simulink model "Simscape_Drone_Model"  (R2025b)
settings: Solver=FixedStepAuto  StartTime=0.0  StopTime=10  RelTol=1e-6  EnableMultiTasking=on
undefined symbols (not defined in the file): Aero_On, Config, P, SimParams, SimscapeParams, X, Y, Z
libraries: sm_lib x89, nesl_utility x71, fl_lib x18, sdl_lib x8, slpidlib x4, batteryecm_lib x1
(part 1 of 5)
settings Model: Creator=Wombat_Simulator  LastModifiedBy=marku
settings SolverCC: ZeroCrossAlgorithm=Adaptive  PositivePriorityOrder=on  AutoInsertRateTranBlk=on
settings DataIOCC: SaveOutput=off  SaveTime=off
settings OptimizationCC: DefaultParameterBehavior=Inlined  EnhancedBackFolding=on  PassReuseOutputArgsAs=Individual arguments  ZeroExternalMemoryAtStartup=off  ZeroInternalMemoryAtStartup=off  MaxStackSize=64  OptimizeBlockOrder=speed  DifferentSizesBufferReuse=on  EfficientTunableParamExpr=on
settings DebuggingCC: IgnoredZcDiagnostic=none  ParameterTunabilityLossMsg=error
settings HardwareCC: ProdBitPerPointer=32.0  ProdBitPerSizeT=32.0  ProdBitPerPtrDiffT=32.0  ProdLargestAtomicInteger=Long  ProdLargestAtomicFloat=Double  ProdWordSize=32.0  ProdHWDeviceType=ARM Compatible->ARM Cortex-A (32-bit)
settings SFSimCC: MATLABDynamicMemAlloc=off
settings RTWCC: SystemTargetFile=ert.tlc  TemplateMakefile=ert_default_tmf  Description=Embedded Coder
settings CodeAppCC: ForceParamTrailComments=on  IgnoreCustomStorageClasses=off  OperatorAnnotations=on  SimulinkDataObjDesc=on  SFDataObjDesc=on  InsertBlockDesc=on
settings ERTTargetCC: ExtModeStaticAlloc=on  InlinedParameterPlacement=Hierarchical  ERTCustomFileTemplate=example_file_process.tlc  SupportNonInlinedSFcns=on
settings ExplorerConfigSet: InternalSimMechanicsExplorerSettings=|
  | <ExplorerConfiguration>
  | 
  |   <canonicalview>default</canonicalview>
  | 
  |   <TilePanel>
  |     <TileInfo>
  |       <Tiles Columns="1" Count="1" Height="1184" Rows="1" Width="2103">
  |         <Row Weight="1"/>
  |         <Column Weight="1"/>
  |         <Tile Height="1" Width="1" X="0" Y="0"/>
  |       </Tiles>
  |     </TileInfo>
  |     <SceneInfo>
  |       <SceneViewer>
  |         <IsThisViewStd>
  |           <IsStandardView>off</IsStandardView>
  |           <StandardViewName>Front</StandardViewName>
  |         </IsThisViewStd>
  |         <BGColor>
  |           <R>1</R>
  |           <G>1</G>
  |           <B>1</B>
  |           <A>1</A>
  |         </BGColor>
  |         <Camera>
  |           <DoPerspective>on</DoPerspective>
  |           <Position>
  |             <X>-0.70406999999999997</X>
  |             <Y>24.994199999999999</Y>
  |             <Z>0.5675</Z>
  |           </Position>
  |           <Center>
  |             <X>-0.56381999999999999</X>
  |             <Y>27.990919999999999</Y>
  |             <Z>-0.43248999999999999</Z>
  |           </Center>
  |           <Up>
  |             <X>0.014783513727254149</X>
  |             <Y>0.31587915334571876</Y>
  |             <Z>0.94868425105694032</Z>
  |           </Up>
  |           <XLim>1.4745942901489864</XLim>
  |           <YLim>1.4745942901489864</YLim>
  |           <ViewLimDist>0.01</ViewLimDist>
  |         </Camera>
  |       </SceneViewer>
  |     </SceneInfo>
  |   </TilePanel>
  | 
  |   <MechEditorPanel>
  |     <GfxPanelCameraMap>
  |       <MapElement CameraMLId="Camera1" GfxPanelIndex="0"/>
  |     </GfxPanelCameraMap>
  |     <Cameras>
  |       <Camera>
  |         <Id>Camera1</Id>
  |         <Value>
  |           <Name>Camera1</Name>
  |           <NativeCamera>
  |             <PositionTrackingFeature>Drone_Mechanics.x6DOF.Camera_frame.F</PositionTrackingFeature>
  |             <CenterTrackingFeature>Drone_Mechanics.x6DOF.CoB</CenterTrackingFeature>
  |             <UpVectorTrackingFeature>Drone_Mechanics.Ground.NED</UpVectorTrackingFeature>
  |             <CenterTrackingOrigin>on</CenterTrackingOrigin>
  |             <UpVectorTrackingDirection>-Z</UpVectorTrackingDirection>
  |           </NativeCamera>
  |         </Value>
  |       </Camera>
  |     </Cameras>
  |     <VideoCreator>
  |       <IncludeTiles>All</IncludeTiles>
  |       <IncludeTime>on</IncludeTime>
  |       <IncludeWorldFrame>off</IncludeWorldFrame>
  |       <PlaybackSpeedRatio>1</PlaybackSpeedRatio>
  |       <FrameRate>30</FrameRate>
  |       <FrameSize>auto</FrameSize>
  |       <VideoFormat>UncompressedAVI</VideoFormat>
  |     </VideoCreator>
  |   </MechEditorPanel>
  | 
  |   <PlaybackSettings>
  |     <PlaybackSpeedFactor>1</PlaybackSpeedFactor>
  |   </PlaybackSettings>
  | 
  | </ExplorerConfiguration>

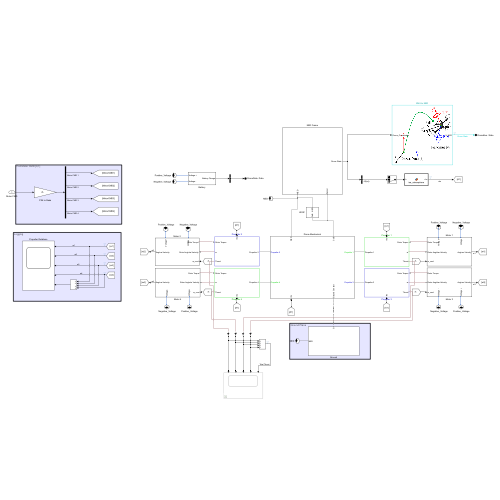
[thumbnail: Simulink's stored preview of the top-level diagram]
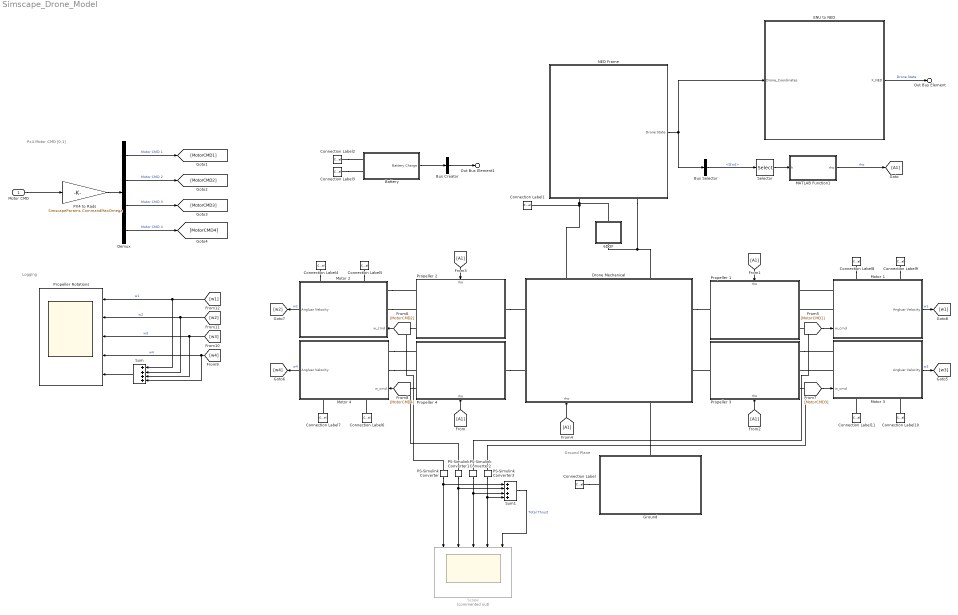
== system Simscape_Drone_Model ==
  note: Logging
  note: Ground Plane
  note: Px4 Motor CMD [0,1]
  Motor CMD : Inport
  6DOF : Subsystem
  Battery : Subsystem
  Bus Creator : BusCreator  Inputs=1
  Bus Selector : BusSelector  OutputSignals=S[m]
  Connection Label : ConnectionLabel  Label=NED
  Connection Label1 : ConnectionLabel  Label=NED
  Connection Label{2,4,6,8,10} (5 alike) : ConnectionLabel  Tag=simrfV2util1/Connection Label  Label=Positive_Voltage
  Connection Label{3,5,7,9,11} (5 alike) : ConnectionLabel  Tag=simrfV2util1/Connection Label  Label=Negative_Voltage
  Demux : Demux
  Drone Mechanical : Subsystem
      settings: PortSchema="{\"entries\":[{\"content\":{\"sides\":[{\"content\":{\"connectorIds\":[\"LConn1\",\"LConn2\"]},\"type\":\"ConnectorPlacement.EquallySpacedRectSide\",\"uuid\":\"5cc608d4-ddbf-4612-8fb9-2660b822e984\"},{\"content\":{\"connectorIds\":[\"RConn1\",\"RConn2\"],\"side\":\"RIGHT\"},\"type\":\"ConnectorPlacement.EquallySpacedRectSide\",\"uuid\":\"5a60fbc0-e4d8-4b3c-ab9e-99a47e43b410\"},{\"content\":{\"connectorIds\":[\"LConn3\",\"LConn4\"],\"side\":\"TOP\"},\"type\":\"ConnectorPlacement.EquallySpacedRectSide\",\"uuid\":\"82070e07-6e43-48ae-84e2-45e211cce44a\"},{\"content\":{\"connectorIds\":[\"In1\",\"RConn3\"],\"side\":\"BOTTOM\"},\"type\":\"ConnectorPlacement.EquallySpacedRectSide\",\"uuid\":\"b93c099a-11e8-4ef2-b906-259b9ea4f5ed\"}]},\"type\":\"ConnectorPlacement.EquallySpacedConnector\",\"uuid\":\"249715e8-12e0-4eae-8212-72e654615a84\"}],\"packageUris\":[\"http://schema.mathworks.com/mf0/Connector/R2020b\"],\"version\":\"1.0\"}"
  ENU to NED : Subsystem
      mask Display: image('World Frame Conversion.png');
  Ground : Subsystem
      settings: PortSchema="{\"entries\":[{\"content\":{\"sides\":[{\"content\":{\"connectorIds\":[\"LConn1\"]},\"type\":\"ConnectorPlacement.EquallySpacedRectSide\",\"uuid\":\"2a080899-5da5-46e1-952c-d17a92ba1a8b\"},{\"content\":{\"side\":\"RIGHT\"},\"type\":\"ConnectorPlacement.EquallySpacedRectSide\",\"uuid\":\"3b513f94-3d5d-4528-8948-7d09eae76d3d\"},{\"content\":{\"connectorIds\":[\"LConn2\"],\"side\":\"TOP\"},\"type\":\"ConnectorPlacement.EquallySpacedRectSide\",\"uuid\":\"f80b446f-13e5-4ac1-9992-a76049c3ec7c\"}]},\"type\":\"ConnectorPlacement.EquallySpacedConnector\",\"uuid\":\"dd2a473b-5f76-4ac8-b09e-9b626a8e8601\"}],\"packageUris\":[\"http://schema.mathworks.com/mf0/Connector/R2020b\"],\"version\":\"1.0\"}"
  MATLAB Function1 : MATLAB Function  TreatAsAtomicUnit=on
  Motor 1 : Subsystem
      settings: PortSchema="{\"entries\":[{\"content\":{\"sides\":[{\"content\":{\"connectorIds\":[\"LConn1\",\"LConn2\",\"In1\"]},\"type\":\"ConnectorPlacement.EquallySpacedRectSide\",\"uuid\":\"33dc3d2f-8968-4f36-a17e-891381f68888\"},{\"content\":{\"connectorIds\":[\"Out1\"],\"side\":\"RIGHT\"},\"type\":\"ConnectorPlacement.EquallySpacedRectSide\",\"uuid\":\"508781b7-b827-4221-88b7-22df8b6754af\"},{\"content\":{\"connectorIds\":[\"LConn3\",\"LConn4\"],\"side\":\"TOP\"},\"type\":\"ConnectorPlacement.EquallySpacedRectSide\",\"uuid\":\"a75d12a6-d4ec-4522-becc-e9bbf7a7aed5\"}]},\"type\":\"ConnectorPlacement.EquallySpacedConnector\",\"uuid\":\"704cc29a-e448-45b3-ab6f-6d8987c901fd\"}],\"packageUris\":[\"http://schema.mathworks.com/mf0/Connector/R2020b\"],\"version\":\"1.0\"}"
  Motor 2 : Subsystem
      settings: PortSchema="{\"entries\":[{\"content\":{\"sides\":[{\"content\":{\"connectorIds\":[\"LConn1\",\"LConn2\",\"In1\"]},\"type\":\"ConnectorPlacement.EquallySpacedRectSide\",\"uuid\":\"ab24fea9-a927-40b5-bce5-f99779c8987a\"},{\"content\":{\"connectorIds\":[\"Out1\"],\"side\":\"RIGHT\"},\"type\":\"ConnectorPlacement.EquallySpacedRectSide\",\"uuid\":\"e5fff93c-3e20-4c5e-b15c-bef5c876d182\"},{\"content\":{\"connectorIds\":[\"LConn3\",\"LConn4\"],\"side\":\"TOP\"},\"type\":\"ConnectorPlacement.EquallySpacedRectSide\",\"uuid\":\"e8b793e7-5ef5-4a63-a387-509c68cd63b8\"}]},\"type\":\"ConnectorPlacement.EquallySpacedConnector\",\"uuid\":\"3d309d3b-67ba-4e78-84bc-eb68d5ca7651\"}],\"packageUris\":[\"http://schema.mathworks.com/mf0/Connector/R2020b\"],\"version\":\"1.0\"}"
  Motor 3 : Subsystem
      settings: PortSchema="{\"entries\":[{\"content\":{\"sides\":[{\"content\":{\"connectorIds\":[\"LConn1\",\"LConn2\",\"In1\"]},\"type\":\"ConnectorPlacement.EquallySpacedRectSide\",\"uuid\":\"33dc3d2f-8968-4f36-a17e-891381f68888\"},{\"content\":{\"connectorIds\":[\"Out1\"],\"side\":\"RIGHT\"},\"type\":\"ConnectorPlacement.EquallySpacedRectSide\",\"uuid\":\"508781b7-b827-4221-88b7-22df8b6754af\"},{\"content\":{\"side\":\"TOP\"},\"type\":\"ConnectorPlacement.EquallySpacedRectSide\",\"uuid\":\"a75d12a6-d4ec-4522-becc-e9bbf7a7aed5\"},{\"content\":{\"connectorIds\":[\"RConn1\",\"RConn2\"],\"side\":\"BOTTOM\"},\"type\":\"ConnectorPlacement.EquallySpacedRectSide\",\"uuid\":\"c496d817-d9a7-4570-9947-2d46969d8890\"}]},\"type\":\"ConnectorPlacement.EquallySpacedConnector\",\"uuid\":\"704cc29a-e448-45b3-ab6f-6d8987c901fd\"}],\"packageUris\":[\"http://schema.mathworks.com/mf0/Connector/R2020b\"],\"version\":\"1.0\"}"
  Motor 4 : Subsystem
      settings: PortSchema="{\"entries\":[{\"content\":{\"sides\":[{\"content\":{\"connectorIds\":[\"In1\",\"LConn1\",\"LConn2\"]},\"type\":\"ConnectorPlacement.EquallySpacedRectSide\",\"uuid\":\"e00824c0-1364-4e77-bc63-912ddc8593ef\"},{\"content\":{\"connectorIds\":[\"Out1\"],\"side\":\"RIGHT\"},\"type\":\"ConnectorPlacement.EquallySpacedRectSide\",\"uuid\":\"0a7636ad-9e2c-497e-9c6a-850c3925dcad\"},{\"content\":{\"connectorIds\":[\"LConn3\",\"LConn4\"],\"side\":\"TOP\"},\"type\":\"ConnectorPlacement.EquallySpacedRectSide\",\"uuid\":\"0b319ad1-75e7-4a0f-96b2-2e5629eeb7ef\"}]},\"type\":\"ConnectorPlacement.EquallySpacedConnector\",\"uuid\":\"157f13eb-3591-4c9f-b2fb-1cc94b60842e\"}],\"packageUris\":[\"http://schema.mathworks.com/mf0/Connector/R2020b\"],\"version\":\"1.0\"}"
  NED Frame : Subsystem
      settings: PortSchema="{\"entries\":[{\"content\":{\"sides\":[{\"content\":{},\"type\":\"ConnectorPlacement.EquallySpacedRectSide\",\"uuid\":\"2f7c4040-ad72-4a4e-bca0-490c9a3edb01\"},{\"content\":{\"connectorIds\":[\"RConn1\",\"RConn2\"],\"side\":\"RIGHT\"},\"type\":\"ConnectorPlacement.EquallySpacedRectSide\",\"uuid\":\"95b4bfac-22e1-4427-9780-ec2091d8174e\"},{\"content\":{\"side\":\"TOP\"},\"type\":\"ConnectorPlacement.EquallySpacedRectSide\",\"uuid\":\"6fc8ef3e-afe1-420d-8beb-cc9354b2a683\"},{\"content\":{\"connectorIds\":[\"Out1\"],\"side\":\"BOTTOM\"},\"type\":\"ConnectorPlacement.EquallySpacedRectSide\",\"uuid\":\"fddcf54a-6ad4-4366-b56a-6290dfac1197\"}]},\"type\":\"ConnectorPlacement.EquallySpacedConnector\",\"uuid\":\"4cba3fee-e392-4a87-a4f1-4e77f5fdcd83\"}],\"packageUris\":[\"http://schema.mathworks.com/mf0/Connector/R2020b\"],\"version\":\"1.0\"}"
  PS-Simulink Converter{,1..3} (4 alike) : nesl_utility/PS-Simulink Converter  PhysicalDomain=network_engine_domain  SubClassName=ps_output  LeftPortType=input  RightPortType=output  PseudoPeriodic=off  Frequencies=[]  VectorFormat=inherit  Unit=inherit  AffineConversion=off
  PX4 to Rads : Gain  Gain=SimscapeParams.CommandMaxOmega
  Propeller 1 : Subsystem
      settings: PortSchema="{\"entries\":[{\"content\":{\"sides\":[{\"content\":{\"connectorIds\":[\"LConn1\"]},\"type\":\"ConnectorPlacement.EquallySpacedRectSide\",\"uuid\":\"a11f93c9-60b9-4980-b5fb-77cb9445bf15\"},{\"content\":{\"connectorIds\":[\"RConn1\",\"RConn2\",\"RConn3\"],\"side\":\"RIGHT\"},\"type\":\"ConnectorPlacement.EquallySpacedRectSide\",\"uuid\":\"b77a8a2e-4ab8-482f-9f6d-d9ab9ea7b696\"},{\"content\":{\"connectorIds\":[\"In1\"],\"side\":\"TOP\"},\"type\":\"ConnectorPlacement.EquallySpacedRectSide\",\"uuid\":\"fb34fa6b-cd57-4423-95d5-7f2443420811\"}]},\"type\":\"ConnectorPlacement.EquallySpacedConnector\",\"uuid\":\"b83f6b43-9a9e-4fc8-9a49-e0da42a3bbd0\"}],\"packageUris\":[\"http://schema.mathworks.com/mf0/Connector/R2020b\"],\"version\":\"1.0\"}"
  Propeller 2 : Subsystem
      settings: PortSchema="{\"entries\":[{\"content\":{\"sides\":[{\"content\":{\"connectorIds\":[\"LConn1\"]},\"type\":\"ConnectorPlacement.EquallySpacedRectSide\",\"uuid\":\"a11f93c9-60b9-4980-b5fb-77cb9445bf15\"},{\"content\":{\"connectorIds\":[\"RConn1\",\"RConn2\",\"RConn3\"],\"side\":\"RIGHT\"},\"type\":\"ConnectorPlacement.EquallySpacedRectSide\",\"uuid\":\"b77a8a2e-4ab8-482f-9f6d-d9ab9ea7b696\"},{\"content\":{\"connectorIds\":[\"In1\"],\"side\":\"TOP\"},\"type\":\"ConnectorPlacement.EquallySpacedRectSide\",\"uuid\":\"fb34fa6b-cd57-4423-95d5-7f2443420811\"},{\"content\":{\"side\":\"BOTTOM\"},\"type\":\"ConnectorPlacement.EquallySpacedRectSide\",\"uuid\":\"49b1b310-8b7b-4cf8-a23d-4dd8be08c88f\"}]},\"type\":\"ConnectorPlacement.EquallySpacedConnector\",\"uuid\":\"b83f6b43-9a9e-4fc8-9a49-e0da42a3bbd0\"}],\"packageUris\":[\"http://schema.mathworks.com/mf0/Connector/R2020b\"],\"version\":\"1.0\"}"
  Propeller 3 : Subsystem
      settings: PortSchema="{\"entries\":[{\"content\":{\"sides\":[{\"content\":{\"connectorIds\":[\"LConn1\"]},\"type\":\"ConnectorPlacement.EquallySpacedRectSide\",\"uuid\":\"a11f93c9-60b9-4980-b5fb-77cb9445bf15\"},{\"content\":{\"connectorIds\":[\"RConn1\",\"RConn2\",\"RConn3\"],\"side\":\"RIGHT\"},\"type\":\"ConnectorPlacement.EquallySpacedRectSide\",\"uuid\":\"b77a8a2e-4ab8-482f-9f6d-d9ab9ea7b696\"},{\"content\":{\"side\":\"TOP\"},\"type\":\"ConnectorPlacement.EquallySpacedRectSide\",\"uuid\":\"fb34fa6b-cd57-4423-95d5-7f2443420811\"},{\"content\":{\"connectorIds\":[\"In1\"],\"side\":\"BOTTOM\"},\"type\":\"ConnectorPlacement.EquallySpacedRectSide\",\"uuid\":\"7aad20ae-aa9d-4d5e-81ba-52dbfeaf9214\"}]},\"type\":\"ConnectorPlacement.EquallySpacedConnector\",\"uuid\":\"b83f6b43-9a9e-4fc8-9a49-e0da42a3bbd0\"}],\"packageUris\":[\"http://schema.mathworks.com/mf0/Connector/R2020b\"],\"version\":\"1.0\"}"
  Propeller 4 : Subsystem
      settings: PortSchema="{\"entries\":[{\"content\":{\"sides\":[{\"content\":{\"connectorIds\":[\"LConn1\"]},\"type\":\"ConnectorPlacement.EquallySpacedRectSide\",\"uuid\":\"a11f93c9-60b9-4980-b5fb-77cb9445bf15\"},{\"content\":{\"connectorIds\":[\"RConn1\",\"RConn2\",\"RConn3\"],\"side\":\"RIGHT\"},\"type\":\"ConnectorPlacement.EquallySpacedRectSide\",\"uuid\":\"b77a8a2e-4ab8-482f-9f6d-d9ab9ea7b696\"},{\"content\":{\"side\":\"TOP\"},\"type\":\"ConnectorPlacement.EquallySpacedRectSide\",\"uuid\":\"fb34fa6b-cd57-4423-95d5-7f2443420811\"},{\"content\":{\"connectorIds\":[\"In1\"],\"side\":\"BOTTOM\"},\"type\":\"ConnectorPlacement.EquallySpacedRectSide\",\"uuid\":\"82da3900-16a5-458e-a9d2-86e2be3a3c24\"}]},\"type\":\"ConnectorPlacement.EquallySpacedConnector\",\"uuid\":\"b83f6b43-9a9e-4fc8-9a49-e0da42a3bbd0\"}],\"packageUris\":[\"http://schema.mathworks.com/mf0/Connector/R2020b\"],\"version\":\"1.0\"}"
  Propeller Rotations : Scope  NumInputPorts=5
      settings: ActiveDisplayYMinimum=-108.37040231135038  ActiveDisplayYMaximum=951.06085463645354
  Scope : Scope  Commented=on  NumInputPorts=5
      settings: ActiveDisplayYMinimum=-798.82748260843846  ActiveDisplayYMaximum=139.02483072762607  DataLoggingVariableName=ScopeData5
  Selector : Selector  InputPortWidth=3  IndexOptions=Index vector (dialog)  Indices=[3]  OutputSizes=1
  Sum : Sum  Inputs=++++
  Sum1 : Sum  Inputs=++++
  Out Bus Element1 : Outport  PortName=DroneData  Element=Data
  Out Bus Element : Outport  Port=2  PortName=DroneBus  Element=State
  wires:
  MATLAB Function1/1(rho) -> [A1]  "rho"
  [A1] -> Propeller 4/1(rho)
  [A1] -> Propeller 1/1(rho)
  [A1] -> Propeller 3/1(rho)
  [A1] -> Propeller 2/1(rho)
  [A1] -> Drone Mechanical/1(rho)
  Sum/1 -> Propeller Rotations/5
  NED Frame/1(Drone State) -> ENU to NED/1(Drone_Coordinates), Bus Selector/1
  Demux/1 -> [MotorCMD1]  "Motor CMD 1"
  [MotorCMD1] -> Motor 1/1(w_cmd)
  Demux/2 -> [MotorCMD2]  "Motor CMD 2"
  [MotorCMD2] -> Motor 2/1(w_cmd)
  Demux/3 -> [MotorCMD3]  "Motor CMD 3"
  [MotorCMD3] -> Motor 3/1(w_cmd)
  Demux/4 -> [MotorCMD4]  "Motor CMD 4"
  [MotorCMD4] -> Motor 4/1(w_cmd)
  Selector/1 -> MATLAB Function1/1(h)
  Bus Selector/1 -> Selector/1  "<S[m]>"
  Battery/1(Battery Charge) -> Bus Creator/1
  Bus Creator/1 -> Out Bus Element1/1
  ENU to NED/1(X_NED) -> Out Bus Element/1  "Drone State"
  PX4 to Rads/1 -> Demux/1
  Motor 3/1(Angluar Velocity) -> [w3]  "w3"
  [w3] -> Propeller Rotations/3, Sum/3  "w3"
  Motor 4/1(Angluar Velocity) -> [w4]  "w4"
  [w4] -> Propeller Rotations/4, Sum/4  "w4"
  Motor 2/1(Angluar Velocity) -> [w2]  "w2"
  [w2] -> Propeller Rotations/2, Sum/2  "w2"
  Motor 1/1(Angluar Velocity) -> [w1]  "w1"
  [w1] -> Propeller Rotations/1, Sum/1  "w1"
  PS-Simulink Converter/1 -> Scope/1, Sum1/1
  PS-Simulink Converter1/1 -> Scope/2, Sum1/2
  PS-Simulink Converter2/1 -> Scope/3, Sum1/3
  PS-Simulink Converter3/1 -> Scope/4, Sum1/4
  Motor CMD/1 -> PX4 to Rads/1
  Sum1/1 -> Scope/5  "Total Thrust"
  connections:
  6DOF/LConn1 -- Connection Label1/LConn1 -- Drone Mechanical/LConn3 -- NED Frame/RConn1
  6DOF/RConn1 -- NED Frame/RConn2 -- Drone Mechanical/LConn4
  Motor 1/LConn2 -- Propeller 1/RConn2
  Propeller 3/LConn1 -- Drone Mechanical/RConn2
  Propeller 3/RConn1 -- Motor 3/LConn1
  Motor 2/LConn1 -- Propeller 2/RConn1
  Connection Label/LConn1 -- Ground/LConn1
  Propeller 2/LConn1 -- Drone Mechanical/LConn1
  Motor 2/LConn2 -- Propeller 2/RConn2
  Propeller 4/LConn1 -- Drone Mechanical/LConn2
  Motor 1/LConn1 -- Propeller 1/RConn1
  Motor 4/LConn1 -- Propeller 4/RConn2
  Ground/LConn2 -- Drone Mechanical/RConn3
  Drone Mechanical/RConn1 -- Propeller 1/LConn1
  Motor 4/LConn2 -- Propeller 4/RConn1
  Motor 3/LConn2 -- Propeller 3/RConn2
  Connection Label2/LConn1 -- Battery/LConn1
  Connection Label3/LConn1 -- Battery/LConn2
  Connection Label4/LConn1 -- Motor 2/LConn4
  Connection Label5/LConn1 -- Motor 2/LConn3
  Connection Label6/LConn1 -- Motor 4/LConn3
  Connection Label7/LConn1 -- Motor 4/LConn4
  Connection Label8/LConn1 -- Motor 1/LConn3
  Connection Label9/LConn1 -- Motor 1/LConn4
  Connection Label11/LConn1 -- Motor 3/RConn1
  Connection Label10/LConn1 -- Motor 3/RConn2
  PS-Simulink Converter/LConn1 -- Propeller 2/RConn3
  PS-Simulink Converter1/LConn1 -- Propeller 4/RConn3
  PS-Simulink Converter2/LConn1 -- Propeller 1/RConn3
  PS-Simulink Converter3/LConn1 -- Propeller 3/RConn3

== system Simscape_Drone_Model/6DOF ==
  6-DOF Joint : sm_lib/Joints/6-DOF Joint  JointMode=Normal  CompositeWrenchDir=FollowerOnBase  CompositeWrenchFrame=BaseFrame  SenseConstraintForce=off  SenseConstraintTorque=off  SenseTotalForce=off  SenseTotalTorque=off  PxPositionTargetSpecify=off  PxPositionTargetPriority=High  PxPositionTargetValue=0  PxPositionTargetValueUnits=m  PxVelocityTargetSpecify=off  PxVelocityTargetPriority=High  PxVelocityTargetValue=0  PxVelocityTargetValueUnits=m/s  PxEquilibriumPosition=0  PxEquilibriumPositionUnits=m  PxSpringStiffness=0  PxSpringStiffnessUnits=N/m  PxDampingCoefficient=0  PxDampingCoefficientUnits=N/(m/s)  PxLowerLimitSpecify=off  PxLowerLimitBound=-1  PxLowerLimitBoundUnits=m  PxLowerLimitStiffness=1e6  PxLowerLimitStiffnessUnits=N/m  PxLowerLimitDamping=1e3  PxLowerLimitDampingUnits=N/(m/s)  PxLowerLimitTransitionRegionWidth=1e-4  PxLowerLimitTransitionRegionWidthUnits=m  PxUpperLimitSpecify=off  PxUpperLimitBound=1  PxUpperLimitBoundUnits=m  PxUpperLimitStiffness=1e6  PxUpperLimitStiffnessUnits=N/m  PxUpperLimitDamping=1e3  PxUpperLimitDampingUnits=N/(m/s)  PxUpperLimitTransitionRegionWidth=1e-4  PxUpperLimitTransitionRegionWidthUnits=m  PxTorqueActuationMode=NoTorque  PxMotionActuationMode=ComputedMotion  PxSensePosition=off  PxSenseVelocity=off  PxSenseAcceleration=off  PxSenseTorqueForce=off  PxSenseLowerLimitTorqueForce=off  PxSenseUpperLimitTorqueForce=off  PyPositionTargetSpecify=off  PyPositionTargetPriority=High  PyPositionTargetValue=0  PyPositionTargetValueUnits=m  PyVelocityTargetSpecify=off  PyVelocityTargetPriority=High  PyVelocityTargetValue=0  PyVelocityTargetValueUnits=m/s  PyEquilibriumPosition=0  PyEquilibriumPositionUnits=m  PySpringStiffness=0  PySpringStiffnessUnits=N/m  PyDampingCoefficient=0  PyDampingCoefficientUnits=N/(m/s)  PyLowerLimitSpecify=off  PyLowerLimitBound=-1  PyLowerLimitBoundUnits=m  PyLowerLimitStiffness=1e6  PyLowerLimitStiffnessUnits=N/m  PyLowerLimitDamping=1e3  PyLowerLimitDampingUnits=N/(m/s)  PyLowerLimitTransitionRegionWidth=1e-4  PyLowerLimitTransitionRegionWidthUnits=m  PyUpperLimitSpecify=off  PyUpperLimitBound=1  PyUpperLimitBoundUnits=m  PyUpperLimitStiffness=1e6  PyUpperLimitStiffnessUnits=N/m  PyUpperLimitDamping=1e3  PyUpperLimitDampingUnits=N/(m/s)  PyUpperLimitTransitionRegionWidth=1e-4  PyUpperLimitTransitionRegionWidthUnits=m  PyTorqueActuationMode=NoTorque  PyMotionActuationMode=ComputedMotion  PySensePosition=off  PySenseVelocity=off  PySenseAcceleration=off  PySenseTorqueForce=off  PySenseLowerLimitTorqueForce=off  PySenseUpperLimitTorqueForce=off  PzPositionTargetSpecify=off  PzPositionTargetPriority=High  PzPositionTargetValue=-500  PzPositionTargetValueUnits=m  PzVelocityTargetSpecify=off  PzVelocityTargetPriority=High  PzVelocityTargetValue=0  PzVelocityTargetValueUnits=m/s  PzEquilibriumPosition=0  PzEquilibriumPositionUnits=m  PzSpringStiffness=0  PzSpringStiffnessUnits=N/m  PzDampingCoefficient=0  PzDampingCoefficientUnits=N/(m/s)  PzLowerLimitSpecify=off  PzLowerLimitBound=-1  PzLowerLimitBoundUnits=m  PzLowerLimitStiffness=1e6  PzLowerLimitStiffnessUnits=N/m  PzLowerLimitDamping=1e3  PzLowerLimitDampingUnits=N/(m/s)  PzLowerLimitTransitionRegionWidth=1e-4  PzLowerLimitTransitionRegionWidthUnits=m  PzUpperLimitSpecify=off  PzUpperLimitBound=1  PzUpperLimitBoundUnits=m  PzUpperLimitStiffness=1e6  PzUpperLimitStiffnessUnits=N/m  PzUpperLimitDamping=1e3  PzUpperLimitDampingUnits=N/(m/s)  PzUpperLimitTransitionRegionWidth=1e-4  PzUpperLimitTransitionRegionWidthUnits=m  PzTorqueActuationMode=NoTorque  PzMotionActuationMode=ComputedMotion  PzSensePosition=off  PzSenseVelocity=off  PzSenseAcceleration=off  PzSenseTorqueForce=off  PzSenseLowerLimitTorqueForce=off  PzSenseUpperLimitTorqueForce=off  SphPositionTargetSpecify=off  SphPositionTargetPriority=High  SphPositionTargetRotationMethod=None  SphPositionTargetFollAlignAxisA=+X  SphPositionTargetBaseAlignAxisA=+Y  SphPositionTargetFollAlignAxisB=+Y  SphPositionTargetBaseAlignAxisB=+Z  SphPositionTargetRotationStandardAxis=+Z  SphPositionTargetRotationAngle=0  SphPositionTargetRotationAngleUnits=deg  SphPositionTargetRotationArbitraryAxis=[0 0 1]  SphPositionTargetRotationSequenceAxes=FollowerAxes  SphPositionTargetRotationSequence=XYX  SphPositionTargetRotationSequenceAngles=[0 0 0]  SphPositionTargetRotationSequenceAnglesUnits=deg  SphPositionTargetRotationMatrix=[1 0 0;0 1 0;0 0 1]  SphPositionTargetQuaternion=[1 0 0 0]  SphVelocityTargetSpecify=off  SphVelocityTargetPriority=High  SphVelocityTargetValue=[0 0 0]  SphVelocityTargetValueUnits=deg/s  SphVelocityTargetInFollowerFrame=on  SphEqPosRotationMethod=None  SphEqPosFollAlignAxisA=+X  SphEqPosBaseAlignAxisA=+Y  SphEqPosFollAlignAxisB=+Y  SphEqPosBaseAlignAxisB=+Z  SphEqPosRotationStandardAxis=+Z  SphEqPosRotationAngle=0  SphEqPosRotationAngleUnits=deg  SphEqPosRotationArbitraryAxis=[0 0 1]  SphEqPosRotationSequenceAxes=FollowerAxes  SphEqPosRotationSequence=XYX  SphEqPosRotationSequenceAngles=[0 0 0]  SphEqPosRotationSequenceAnglesUnits=deg  SphEqPosRotationMatrix=[1 0 0;0 1 0;0 0 1]  SphEqPosQuaternion=[1 0 0 0]  SphSpringStiffness=0  SphSpringStiffnessUnits=N*m/deg  SphDampingCoefficient=0  SphDampingCoefficientUnits=N*m/(deg/s)  SphLowerLimitSpecify=off  SphLowerLimitBound=15  SphLowerLimitBoundUnits=deg  SphLowerLimitStiffness=1e4  SphLowerLimitStiffnessUnits=N*m/deg  SphLowerLimitDamping=10  SphLowerLimitDampingUnits=N*m/(deg/s)  SphLowerLimitTransitionRegionWidth=0.1  SphLowerLimitTransitionRegionWidthUnits=deg  SphUpperLimitSpecify=off  SphUpperLimitBound=45  SphUpperLimitBoundUnits=deg  SphUpperLimitStiffness=1e4  SphUpperLimitStiffnessUnits=N*m/deg  SphUpperLimitDamping=10  SphUpperLimitDampingUnits=N*m/(deg/s)  SphUpperLimitTransitionRegionWidth=0.1  SphUpperLimitTransitionRegionWidthUnits=deg  SphTorqueActuationMode=NoTorque  SphActuateTorqueX=off  SphActuateTorqueY=off  SphActuateTorqueZ=off  SphActuateTorque=off  SphActuationFrame=BaseFrame  SphSensePosition=off  SphSenseVelocityX=off  SphSenseVelocityY=off  SphSenseVelocityZ=off  SphSenseVelocity=off  SphSenseAccelerationX=off  SphSenseAccelerationY=off  SphSenseAccelerationZ=off  SphSenseAcceleration=off  SphSenseLowerLimitTorqueMag=off  SphSenseUpperLimitTorqueMag=off  SphSensingFrame=BaseFrame
  Camera frame : sm_lib/Frames and Transforms/Rigid Transform  Commented=on  RotationMethod=RotationSequence  FollAlignAxisA=+X  BaseAlignAxisA=+Y  FollAlignAxisB=+Y  BaseAlignAxisB=+Z  RotationStandardAxis=+Z  RotationAngle=0  RotationAngleUnits=deg  RotationArbitraryAxis=[0 0 1]  RotationSequenceAxes=BaseAxes  RotationSequence=XYZ  RotationSequenceAngles=[0 0 0]  RotationSequenceAnglesUnits=deg  RotationMatrix=[1 0 0;0 1 0;0 0 1]  Quaternion=[1 0 0 0]  TranslationMethod=Cartesian  TranslationCartesianOffset=[-5 0 -2]  TranslationCartesianOffsetUnits=m  TranslationStandardAxis=+Z  TranslationStandardOffset=0  TranslationStandardOffsetUnits=m  TranslationROffset=0  TranslationROffsetUnits=m  TranslationThetaOffset=0  TranslationThetaOffsetUnits=deg  TranslationZOffset=0  TranslationZOffsetUnits=m
  Inertia1 : sm_lib/Body Elements/Inertia  Commented=on  InertiaType=PointMass  Mass=0.00000001  MassUnits=kg  CenterOfMass=[0 0 0]  CenterOfMassUnits=m  MomentsOfInertia=[1 1 1]  MomentsOfInertiaUnits=kg*m^2  ProductsOfInertia=[0 0 0]  ProductsOfInertiaUnits=kg*m^2  GraphicType=None  MarkerShape=Inertia  MarkerSize=20  GraphicVisPropType=SimpleVisualProperties  GraphicDiffuseColor=[0.5 0.5 0.5]  GraphicOpacity=1  GraphicSpecularColor=[0.5 0.5 0.5 1.0]  GraphicAmbientColor=[0.15 0.15 0.15 1.0]  GraphicEmissiveColor=[0.0 0.0 0.0 1.0]  GraphicShininess=75
  NED : PMIOPort  Side=Left
  CoB : PMIOPort  Port=2  Side=Right
  connections:
  Inertia1/RConn1 -- Camera frame/RConn1
  Camera frame/LConn1 -- 6-DOF Joint/RConn1 -- CoB/RConn1
  6-DOF Joint/LConn1 -- NED/RConn1

== system Simscape_Drone_Model/Battery ==
  Battery1 : batteryecm_lib/Battery  Vnom=21.6 V  prm_dir=simscape.enum.battery.prm_dir.disabled  R1_dis=2 Ohm  R1_ch=2 Ohm  R1=0.01 Ohm  prm_AH=simscape.enum.battery.prm_AH.infinite  AH=50 A*hr  V1=11.5 V  AH1=25 A*hr  prm_R2=simscape.enum.battery.prm_R2.disabled  R2=2000 Ohm  Tmeas=298.15 K  charge_measurement_port=simscape.enum.battery.enable.yes  prm_dyn=simscape.enum.battery.prm_dyn.off  Rp1=0.005 Ohm  tau1=30 s  Rp2=0.005 Ohm  tau2=30 s  Rp3=0.005 Ohm  tau3=30 s  Rp4=0.005 Ohm  tau4=30 s  Rp5=0.005 Ohm  tau5=30 s  prm_fade=simscape.enum.battery.prm_fade.disabled  N_fade=100  AH_fade=45 A*hr  R1_fade=2.02 Ohm  R1_ch_fade=2.02 Ohm  V1_fade=10.35 V  prm_age=simscape.enum.battery.prm_age.disabled  prm_age_OCV=simscape.enum.battery.prm_age_OCV.OCV  OCV_age=0.9  SOC_age=60  Tmeas_age=298.15 K  delta_time_age_vec=[0] d  temperature_age_vec=[273] K  OCV_scaling_age=2.2134e6  OCV_offset_age=1.632e6  temp_exp_age=0.515833569 V  t_exp_age=0.75  Vnom_T2=12 V  R1_T2=2.2 Ohm  R1_T2_dis=2.2 Ohm  R1_T2_ch=2.2 Ohm  V1_T2=11.4 V  R2_T2=2200 Ohm  Rp1_T2=0.005 Ohm  tau1_T2=30 s  Rp2_T2=0.005 Ohm  tau2_T2=30 s  Rp3_T2=0.005 Ohm  tau3_T2=30 s  Rp4_T2=0.005 Ohm  tau4_T2=30 s  Rp5_T2=0.005 Ohm  tau5_T2=30 s  Tmeas2=273.15 K  thermal_port=simscape.enum.thermaleffects.omit  thermal_mass=30000 J/K  i_specify=off  i_priority=None  i=0 A  i_nominal_specify=off  i_nominal_value=1  i_nominal_unit=A  v_specify=off  v_priority=None  v=0 V  v_nominal_specify=off  v_nominal_value=1  v_nominal_unit=V  charge_specify=off  charge_priority=High  charge=50 A*hr  charge_nominal_specify=off  charge_nominal_value=1  charge_nominal_unit=A*hr  num_cycles_specify=off  num_cycles_priority=High  num_cycles=0  num_cycles_nominal_specify=off  num_cycles_nominal_value=1  num_cycles_nominal_unit=1  temperature_specify=off  temperature_priority=High  temperature=298.15 K  temperature_nominal_specify=off  temperature_nominal_value=1  temperature_nominal_unit=K
      settings: InternalSimscapePortConfiguration="{\"Bottom\":[],\"Left\":[{\"id\":\"p\",\"label\":\"+\",\"type\":\"foundation.electrical.electrical\"},{\"id\":\"q\",\"label\":\"q\",\"type\":\"output\"}],\"Right\":[{\"id\":\"n\",\"label\":\"-\",\"type\":\"foundation.electrical.electrical\"}],\"Top\":[]}"
  Electrical Reference : fl_lib/Electrical/Electrical Elements/Electrical Reference
  PS-Simulink Converter : nesl_utility/PS-Simulink Converter  PhysicalDomain=network_engine_domain  SubClassName=ps_output  LeftPortType=input  RightPortType=output  PseudoPeriodic=off  Frequencies=[]  VectorFormat=inherit  Unit=inherit  AffineConversion=off
  PS-Simulink Converter1 : nesl_utility/PS-Simulink Converter  PhysicalDomain=network_engine_domain  SubClassName=ps_output  LeftPortType=input  RightPortType=output  PseudoPeriodic=off  Frequencies=[]  VectorFormat=inherit  Unit=inherit  AffineConversion=off
  Scope : Scope
      settings: ActiveDisplayYMinimum=21.175481985714523  ActiveDisplayYMaximum=21.647172881569247
  Voltage Sensor : fl_lib/Electrical/Electrical Sensors/Voltage Sensor
  Voltage + : PMIOPort  Side=Left
  Voltage - : PMIOPort  Port=2  Side=Left
  Battery Charge : Outport
  wires:
  PS-Simulink Converter/1 -> Scope/1
  PS-Simulink Converter1/1 -> Battery Charge/1
  connections:
  PS-Simulink Converter/LConn1 -- Voltage Sensor/RConn1
  Battery1/LConn1 -- Voltage Sensor/LConn1 -- Voltage +/RConn1
  Battery1/RConn1 -- Voltage -/RConn1 -- Voltage Sensor/RConn2 -- Electrical Reference/LConn1
  Battery1/LConn2 -- PS-Simulink Converter1/LConn1

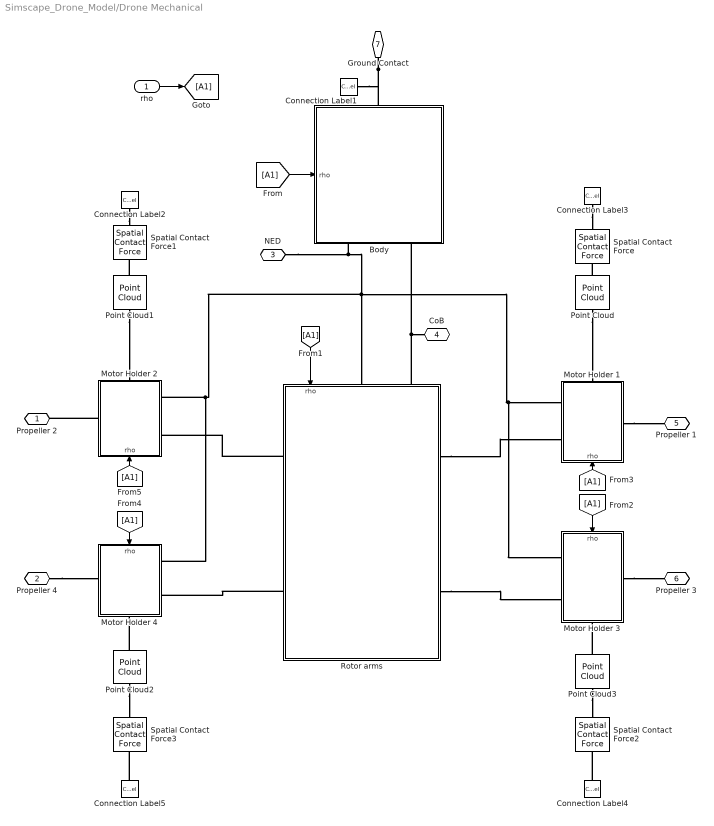
== system Simscape_Drone_Model/Drone Mechanical ==
  rho : Inport
  Body : Subsystem
      settings: PortSchema="{\"entries\":[{\"content\":{\"sides\":[{\"content\":{\"connectorIds\":[\"LConn1\"]},\"type\":\"ConnectorPlacement.EquallySpacedRectSide\",\"uuid\":\"eafa4ad9-9f6d-4883-93a7-4653add6d79e\"},{\"content\":{\"connectorIds\":[\"RConn1\",\"RConn2\"],\"side\":\"RIGHT\"},\"type\":\"ConnectorPlacement.EquallySpacedRectSide\",\"uuid\":\"9303d811-4b4b-4772-90ea-d0407e17ab5a\"},{\"content\":{\"connectorIds\":[\"In1\"],\"side\":\"TOP\"},\"type\":\"ConnectorPlacement.EquallySpacedRectSide\",\"uuid\":\"296d3f1d-3dd2-41a2-b4be-cbb0139b1c5a\"},{\"content\":{\"side\":\"BOTTOM\"},\"type\":\"ConnectorPlacement.EquallySpacedRectSide\",\"uuid\":\"db543621-34ee-4e75-a25d-c010b66f2eda\"}]},\"type\":\"ConnectorPlacement.EquallySpacedConnector\",\"uuid\":\"34ab0763-b5b5-4abc-88cc-a4cc11a4bce2\"}],\"packageUris\":[\"http://schema.mathworks.com/mf0/Connector/R2020b\"],\"version\":\"1.0\"}"
  Connection Label{1..5} (5 alike) : ConnectionLabel  Label=Ground
  Motor Holder 1 : Subsystem
      settings: PortSchema="{\"entries\":[{\"content\":{\"sides\":[{\"content\":{\"connectorIds\":[\"LConn1\",\"LConn2\"]},\"type\":\"ConnectorPlacement.EquallySpacedRectSide\",\"uuid\":\"d3ec4a2e-ccb4-40a1-80e4-1a956df35da0\"},{\"content\":{\"connectorIds\":[\"RConn1\"],\"side\":\"RIGHT\"},\"type\":\"ConnectorPlacement.EquallySpacedRectSide\",\"uuid\":\"37090704-0417-45f9-ad2c-7dab35db7d02\"},{\"content\":{\"connectorIds\":[\"LConn3\"],\"side\":\"TOP\"},\"type\":\"ConnectorPlacement.EquallySpacedRectSide\",\"uuid\":\"c7444435-31c3-4cd2-a94b-9ada716925cd\"},{\"content\":{\"connectorIds\":[\"In1\"],\"side\":\"BOTTOM\"},\"type\":\"ConnectorPlacement.EquallySpacedRectSide\",\"uuid\":\"a22718fd-cbcb-4bc2-bb33-1f3bb561ecba\"}]},\"type\":\"ConnectorPlacement.EquallySpacedConnector\",\"uuid\":\"fe7a8740-e461-4d7f-ab39-6d0769c04c90\"}],\"packageUris\":[\"http://schema.mathworks.com/mf0/Connector/R2020b\"],\"version\":\"1.0\"}"
  Motor Holder 2 : Subsystem
      settings: PortSchema="{\"entries\":[{\"content\":{\"sides\":[{\"content\":{\"connectorIds\":[\"LConn1\",\"LConn2\"]},\"type\":\"ConnectorPlacement.EquallySpacedRectSide\",\"uuid\":\"d3ec4a2e-ccb4-40a1-80e4-1a956df35da0\"},{\"content\":{\"connectorIds\":[\"RConn1\"],\"side\":\"RIGHT\"},\"type\":\"ConnectorPlacement.EquallySpacedRectSide\",\"uuid\":\"37090704-0417-45f9-ad2c-7dab35db7d02\"},{\"content\":{\"connectorIds\":[\"LConn3\"],\"side\":\"TOP\"},\"type\":\"ConnectorPlacement.EquallySpacedRectSide\",\"uuid\":\"c7444435-31c3-4cd2-a94b-9ada716925cd\"},{\"content\":{\"connectorIds\":[\"In1\"],\"side\":\"BOTTOM\"},\"type\":\"ConnectorPlacement.EquallySpacedRectSide\",\"uuid\":\"fed292c2-8921-4dad-a433-f1084b2195d3\"}]},\"type\":\"ConnectorPlacement.EquallySpacedConnector\",\"uuid\":\"fe7a8740-e461-4d7f-ab39-6d0769c04c90\"}],\"packageUris\":[\"http://schema.mathworks.com/mf0/Connector/R2020b\"],\"version\":\"1.0\"}"
  Motor Holder 3 : Subsystem
      settings: PortSchema="{\"entries\":[{\"content\":{\"sides\":[{\"content\":{\"connectorIds\":[\"LConn1\",\"LConn2\"]},\"type\":\"ConnectorPlacement.EquallySpacedRectSide\",\"uuid\":\"d3ec4a2e-ccb4-40a1-80e4-1a956df35da0\"},{\"content\":{\"connectorIds\":[\"RConn1\"],\"side\":\"RIGHT\"},\"type\":\"ConnectorPlacement.EquallySpacedRectSide\",\"uuid\":\"37090704-0417-45f9-ad2c-7dab35db7d02\"},{\"content\":{\"connectorIds\":[\"In1\"],\"side\":\"TOP\"},\"type\":\"ConnectorPlacement.EquallySpacedRectSide\",\"uuid\":\"c7444435-31c3-4cd2-a94b-9ada716925cd\"},{\"content\":{\"connectorIds\":[\"RConn2\"],\"side\":\"BOTTOM\"},\"type\":\"ConnectorPlacement.EquallySpacedRectSide\",\"uuid\":\"0bb0b4a1-4aad-4457-bf67-affc5c4927c6\"}]},\"type\":\"ConnectorPlacement.EquallySpacedConnector\",\"uuid\":\"fe7a8740-e461-4d7f-ab39-6d0769c04c90\"}],\"packageUris\":[\"http://schema.mathworks.com/mf0/Connector/R2020b\"],\"version\":\"1.0\"}"
  Motor Holder 4 : Subsystem
      settings: PortSchema="{\"entries\":[{\"content\":{\"sides\":[{\"content\":{\"connectorIds\":[\"LConn1\",\"LConn2\"]},\"type\":\"ConnectorPlacement.EquallySpacedRectSide\",\"uuid\":\"d3ec4a2e-ccb4-40a1-80e4-1a956df35da0\"},{\"content\":{\"connectorIds\":[\"RConn1\"],\"side\":\"RIGHT\"},\"type\":\"ConnectorPlacement.EquallySpacedRectSide\",\"uuid\":\"37090704-0417-45f9-ad2c-7dab35db7d02\"},{\"content\":{\"connectorIds\":[\"In1\"],\"side\":\"TOP\"},\"type\":\"ConnectorPlacement.EquallySpacedRectSide\",\"uuid\":\"c7444435-31c3-4cd2-a94b-9ada716925cd\"},{\"content\":{\"connectorIds\":[\"RConn2\"],\"side\":\"BOTTOM\"},\"type\":\"ConnectorPlacement.EquallySpacedRectSide\",\"uuid\":\"4a250118-2daa-49a6-8e90-ca75e0b9d2b5\"}]},\"type\":\"ConnectorPlacement.EquallySpacedConnector\",\"uuid\":\"fe7a8740-e461-4d7f-ab39-6d0769c04c90\"}],\"packageUris\":[\"http://schema.mathworks.com/mf0/Connector/R2020b\"],\"version\":\"1.0\"}"
  Point Cloud{,1..3} (4 alike) : sm_lib/Curves and Surfaces/Point Cloud  CoordinatesMatrix=SimscapeParams.MotorSurfacePoints  CoordinatesMatrixUnits=m  GraphicType=None  GraphicSphereRadius=1e-2  GraphicSphereRadiusUnits=m  GraphicVisPropType=SimpleVisualProperties  GraphicDiffuseColor=[0.5 0.5 0.5]  GraphicOpacity=1  GraphicSpecularColor=[0.5 0.5 0.5 1.0]  GraphicAmbientColor=[0.15 0.15 0.15 1.0]  GraphicEmissiveColor=[0.0 0.0 0.0 1.0]  GraphicShininess=75
  Rotor arms : Subsystem
      settings: PortSchema="{\"entries\":[{\"content\":{\"sides\":[{\"content\":{\"connectorIds\":[\"LConn1\",\"LConn2\"]},\"type\":\"ConnectorPlacement.EquallySpacedRectSide\",\"uuid\":\"1a6cdd76-3e86-40cc-a8b8-1b2852a69cf7\"},{\"content\":{\"connectorIds\":[\"RConn1\",\"RConn2\"],\"side\":\"RIGHT\"},\"type\":\"ConnectorPlacement.EquallySpacedRectSide\",\"uuid\":\"946eb998-e646-4a55-aabb-8736804e1b93\"},{\"content\":{\"connectorIds\":[\"In1\",\"LConn3\",\"LConn4\"],\"side\":\"TOP\"},\"type\":\"ConnectorPlacement.EquallySpacedRectSide\",\"uuid\":\"ae865b22-9b66-413b-b43a-0fb2df2ce8a5\"}]},\"type\":\"ConnectorPlacement.EquallySpacedConnector\",\"uuid\":\"ebfaf115-33d0-4706-a700-a30f7a6f854e\"}],\"packageUris\":[\"http://schema.mathworks.com/mf0/Connector/R2020b\"],\"version\":\"1.0\"}"
  Spatial Contact Force{,1..3} (4 alike) : sm_lib/Forces and Torques/Spatial Contact Force  SenseSeparationDistance=off  NormalForceType=SmoothSpringDamper  NormalStiffness=2.5e5  NormalStiffnessUnits=N/m  NormalDamping=250  NormalDampingUnits=N/(m/s)  NormalTransitionRegionWidth=1e-4  NormalTransitionRegionWidthUnits=m  FrictionType=None  CoefficientOfStaticFriction=0.5  CoefficientOfDynamicFriction=0.3  FrictionalCriticalVelocity=1e-4  FrictionalCriticalVelocityUnits=m/s  SenseContactSignal=off  SensePenetrationDepth=off  SenseNormalVelocity=off  SenseTangentialVelocity=off  SensingForceTorqueDirection=BaseOnFollower  SensingForceTorqueResolutionFrame=ContactFrame  SenseNormalForce=off  SenseNormalForceMagnitude=off  SenseNormalTorque=off  SenseFrictionalForce=off  SenseFrictionalForceMagnitude=off  SenseFrictionalTorque=off  SenseTotalForce=off  SenseTotalTorque=off  SenseContactBaseRotation=off  SenseContactBaseTranslation=off  SenseContactFollowerRotation=off  SenseContactFollowerTranslation=off  ZeroCrossDetectContactStartAndEnd=off
  Propeller 2 : PMIOPort  Side=Left
  Propeller 4 : PMIOPort  Port=2  Side=Left
  NED : PMIOPort  Port=3  Side=Left
  CoB : PMIOPort  Port=4  Side=Left
  Propeller 1 : PMIOPort  Port=5  Side=Right
  Propeller 3 : PMIOPort  Port=6  Side=Right
  Ground Contact : PMIOPort  Port=7  Side=Right
  wires:
  [A1] -> Motor Holder 3/1(rho)
  [A1] -> Motor Holder 1/1(rho)
  [A1] -> Motor Holder 2/1(rho)
  [A1] -> Motor Holder 4/1(rho)
  [A1] -> Rotor arms/1(rho)
  [A1] -> Body/1(rho)
  rho/1 -> [A1]
  connections:
  Connection Label5/LConn1 -- Spatial Contact Force3/RConn1
  Connection Label4/LConn1 -- Spatial Contact Force2/RConn1
  Ground Contact/RConn1 -- Body/LConn1 -- Connection Label1/LConn1
  Connection Label3/LConn1 -- Spatial Contact Force/RConn1
  Connection Label2/LConn1 -- Spatial Contact Force1/RConn1
  Body/RConn1 -- NED/RConn1 -- Rotor arms/LConn3 -- Motor Holder 2/LConn1 -- Motor Holder 4/LConn1 -- Motor Holder 1/LConn1 -- Motor Holder 3/LConn1
  Rotor arms/RConn2 -- Motor Holder 3/LConn2
  Rotor arms/RConn1 -- Motor Holder 1/LConn2
  Rotor arms/LConn1 -- Motor Holder 2/LConn2
  Rotor arms/LConn2 -- Motor Holder 4/LConn2
  Point Cloud1/LConn1 -- Motor Holder 2/LConn3
  Point Cloud2/LConn1 -- Motor Holder 4/RConn2
  Propeller 4/RConn1 -- Motor Holder 4/RConn1
  Point Cloud2/RConn1 -- Spatial Contact Force3/LConn1
  Point Cloud3/RConn1 -- Spatial Contact Force2/LConn1
  Point Cloud/RConn1 -- Spatial Contact Force/LConn1
  Point Cloud1/RConn1 -- Spatial Contact Force1/LConn1
  Point Cloud/LConn1 -- Motor Holder 1/LConn3
  Point Cloud3/LConn1 -- Motor Holder 3/RConn2
  Motor Holder 1/RConn1 -- Propeller 1/RConn1
  Motor Holder 3/RConn1 -- Propeller 3/RConn1
  Motor Holder 2/RConn1 -- Propeller 2/RConn1
  CoB/RConn1 -- Rotor arms/LConn4 -- Body/RConn2

== system Simscape_Drone_Model/ENU to NED ==
  Drone_Coordinates : Inport
  Bus Selector : BusSelector  OutputSignals=S[m],S_dot [m/s],S_ddot [m/s^2],Omega [rads/s],Eta [rads],Orientation
  MATLAB Function : MATLAB Function  TreatAsAtomicUnit=on
  S_NED : Scope  Commented=on  NumInputPorts=8
      settings: ActiveDisplayString=6  ActiveDisplayYMinimum=-0.15297724345009411  ActiveDisplayYMaximum=1.1281085826055675  DataLoggingVariableName=ScopeData8
  X_ned : BusCreator  Inputs=6
  X_NED : Outport
  wires:
  Drone_Coordinates/1 -> Bus Selector/1
  MATLAB Function/2(Sdot_ned) -> S_NED/2, X_ned/2  "Sdot_NED"
  MATLAB Function/1(S_ned) -> X_ned/1, S_NED/1  "S_NED"
  MATLAB Function/6(Eta_ned) -> S_NED/5, X_ned/4  "Eta_NED"
  MATLAB Function/3(Sddot_ned) -> X_ned/3, S_NED/3  "Sddot_NED"
  X_ned/1 -> X_NED/1  "X_NED"
  MATLAB Function/7(R_ned) -> S_NED/6  "R_ned"
  Bus Selector/1 -> MATLAB Function/1(S_base)  "<S[m]>"
  Bus Selector/2 -> MATLAB Function/2(Sdot_base)  "<S_dot [m/s]>"
  Bus Selector/3 -> MATLAB Function/3(Sddot_base)  "<S_ddot [m/s^2]>"
  Bus Selector/4 -> MATLAB Function/4(Omega_base)  "<Omega [rads/s]>"
  Bus Selector/5 -> MATLAB Function/5(Eta_in)  "<Eta [rads]>"
  Bus Selector/6 -> MATLAB Function/6(R_raw)  "<Orientation>"
  MATLAB Function/5(Omega_nav_ned) -> S_NED/7, X_ned/5  "Omega_nav_ned"
  MATLAB Function/8(R_ned_to_frd) -> X_ned/6, S_NED/8
  MATLAB Function/4(Omega_frd) -> S_NED/4  "Omega_nav_ned"

== system Simscape_Drone_Model/Ground ==
  GroundPlane : sm_lib/Body Elements/Brick Solid  Commented=on  BrickDimensions=[2 2 0.1]  BrickDimensionsUnits=m  ExportEntireGeometry=off  InertiaType=CalculateFromGeometry  BasedOnType=Density  Density=1000  DensityUnits=kg/m^3  Mass=1  MassUnits=kg  CenterOfMass=[0 0 0]  CenterOfMassUnits=m  MomentsOfInertia=[1 1 1]  MomentsOfInertiaUnits=kg*m^2  ProductsOfInertia=[0 0 0]  ProductsOfInertiaUnits=kg*m^2  GraphicType=FromGeometry  MarkerShape=Sphere  MarkerSize=10  GraphicVisPropType=SimpleVisualProperties  GraphicDiffuseColor=[0.5 0.5 0.5]  GraphicOpacity=1  GraphicSpecularColor=[0.5 0.5 0.5 1.0]  GraphicAmbientColor=[0.15 0.15 0.15 1.0]  GraphicEmissiveColor=[0.0 0.0 0.0 1.0]  GraphicShininess=75  DoExposeReferenceFrame=on  SerializedFrames=<Frames/>
  Infinite Plane : sm_lib/Curves and Surfaces/Infinite Plane  GraphicType=Rectangle  GraphicPlaneWidth=200  GraphicPlaneWidthUnits=m  GraphicPlaneHeight=200  GraphicPlaneHeightUnits=m  GraphicVisPropType=SimpleVisualProperties  GraphicDiffuseColor=[1 0.6667 1]  GraphicOpacity=0.4  GraphicSpecularColor=[0.5 0.5 0.5 1.0]  GraphicAmbientColor=[0.15 0.15 0.15 1.0]  GraphicEmissiveColor=[0.0 0.0 0.0 1.0]  GraphicShininess=75
  Rigid Transform : sm_lib/Frames and Transforms/Rigid Transform  RotationMethod=StandardAxis  FollAlignAxisA=+X  BaseAlignAxisA=+Y  FollAlignAxisB=+Y  BaseAlignAxisB=+Z  RotationStandardAxis=+Y  RotationAngle=180  RotationAngleUnits=deg  RotationArbitraryAxis=[0 0 1]  RotationSequenceAxes=FollowerAxes  RotationSequence=XYX  RotationSequenceAngles=[0 0 0]  RotationSequenceAnglesUnits=deg  RotationMatrix=[1 0 0;0 1 0;0 0 1]  Quaternion=[1 0 0 0]  TranslationMethod=StandardAxis  TranslationCartesianOffset=[0 0 0]  TranslationCartesianOffsetUnits=m  TranslationStandardAxis=+Z  TranslationStandardOffset=0.1  TranslationStandardOffsetUnits=m  TranslationROffset=0  TranslationROffsetUnits=m  TranslationThetaOffset=0  TranslationThetaOffsetUnits=deg  TranslationZOffset=0  TranslationZOffsetUnits=m
  NED : PMIOPort  Side=Left
  G : PMIOPort  Port=2  Side=Left
  connections:
  Infinite Plane/RConn1 -- G/RConn1
  GroundPlane/RConn1 -- NED/RConn1 -- Rigid Transform/LConn1
  Infinite Plane/LConn1 -- Rigid Transform/RConn1

== system Simscape_Drone_Model/Motor 1 ==
  w_cmd : Inport
  Mechanical Rotational Reference : fl_lib/Mechanical/Rotational Elements/Mechanical Rotational Reference
  Mechanical Rotational Reference1 : fl_lib/Mechanical/Rotational Elements/Mechanical Rotational Reference
  Motor 1 : sdl_lib/Engines & Motors/Motor & Drive  torque_max=SimscapeParams.MotorMaxTorque N*m  power_max="SimscapeParams.MotorMaxPower  W"  Tc="SimscapeParams.MotorTorqueControlTimeConstant  s"  eff=SimscapeParams.MotorEfficiency  w_eff="SimscapeParams.MotorEfficiencyMeasurementSpeed  rpm"  T_eff=SimscapeParams.MotorEfficiencyMeasurementTorque N*m  thermal_port=simscape.enum.thermaleffects.omit  thermal_mass=100 J/K  temperature_specify=off  temperature_priority=High  temperature=300 K  temperature_nominal_specify=off  temperature_nominal_value=1  temperature_nominal_unit=K
      settings: InternalSimscapePortConfiguration="{\"Bottom\":[],\"Left\":[{\"id\":\"Vp\",\"label\":\"+\",\"type\":\"foundation.electrical.electrical\"},{\"id\":\"Tr\",\"label\":\"Tr\",\"type\":\"input\"},{\"id\":\"R\",\"label\":\"R\",\"type\":\"foundation.mechanical.rotational.rotational\"}],\"Right\":[{\"id\":\"Vm\",\"label\":\"-\",\"type\":\"foundation.electrical.electrical\"},{\"id\":\"Omega\",\"label\":\"w\",\"type\":\"output\"},{\"id\":\"C\",\"label\":\"C\",\"type\":\"foundation.mechanical.rotational.rotational\"}],\"Top\":[]}"
  PS-Simulink Converter4 : nesl_utility/PS-Simulink Converter  PhysicalDomain=network_engine_domain  SubClassName=ps_output  LeftPortType=input  RightPortType=output  PseudoPeriodic=off  Frequencies=[]  VectorFormat=inherit  Unit=inherit  AffineConversion=off
  Rotational Multibody Interface : fl_lib/Mechanical/Multibody Interfaces/Rotational Multibody Interface
  Simulink-PS Converter : nesl_utility/Simulink-PS Converter  PhysicalDomain=network_engine_domain  SubClassName=ps_input  LeftPortType=input  RightPortType=output  PseudoPeriodic=off  Frequencies=[]  NoiseDistribution=none  NoiseParameters=[]  Unit=1  AffineConversion=off  FilteringAndDerivatives=provide  SimscapeFilterOrder=1  InputFilterTimeConstant=0.001  UdotUserProvided=0
  Sum : Sum  Inputs=|+-
  Thrust Controller : slpidlib/PID Controller  Controller=PI  Form=Parallel  TimeDomain=Continuous-time  UseExternalTs=off  SampleTime=-1  IntegratorMethod=Forward Euler  FilterMethod=Forward Euler  ControllerParametersSource=internal  P=SimscapeParams.MotorKp  I=SimscapeParams.MotorKi  UseKiTs=off  D=0.01  UseExternalDerivativeSource=off  N=100  UseFilter=on  TunerSelectOption=Transfer Function Based (PID Tuner App)  InitialConditionSource=internal  InitialConditionForIntegrator=0  InitialConditionForFilter=0  DifferentiatorICPrevScaledInput=0  ExternalReset=none  TrackingMode=off  Kt=1  LimitOutput=on  SatLimitsSource=internal  UpperSaturationLimit=0.25  LowerSaturationLimit=-0.25  LinearizeAsGain=on  AntiWindupMode=clamping  Kb=1  LimitIntegrator=off  UpperIntegratorSaturationLimit=inf  LowerIntegratorSaturationLimit=-inf  POutMin=[]  POutMax=[]  IOutMin=[]  IOutMax=[]  DOutMin=[]  DOutMax=[]  NOutMin=[]  NOutMax=[]  SumOutMin=[]  SumOutMax=[]  SaturationOutMin=[]  SaturationOutMax=[]  PParamMin=[]  PParamMax=[]  IParamMin=[]  IParamMax=[]  DParamMin=[]  DParamMax=[]  NParamMin=[]  NParamMax=[]  KbParamMin=[]  KbParamMax=[]  KtParamMin=[]  KtParamMax=[]  KbOutMin=[]  KbOutMax=[]  KtOutMin=[]  KtOutMax=[]  IntegratorOutMin=[]  IntegratorOutMax=[]  FilterOutMin=[]  FilterOutMax=[]  SumI1OutMin=[]  SumI1OutMax=[]  SumI2OutMin=[]  SumI2OutMax=[]  SumI3OutMin=[]  SumI3OutMax=[]  SumI4OutMin=[]  SumI4OutMax=[]  SumDOutMin=[]  SumDOutMax=[]  DifferentiatorOutMin=[]  DifferentiatorOutMax=[]  FilterDiffOutCoefMin=[]  FilterDiffOutCoefMax=[]  ReciprocalOutMin=[]  ReciprocalOutMax=[]  SumDenOutMin=[]  SumDenOutMax=[]  SumNumOutMin=[]  SumNumOutMax=[]  DivideOutMin=[]  DivideOutMax=[]  UdiffTsProdOutMin=[]  UdiffTsProdOutMax=[]  NTsProdOutMin=[]  NTsProdOutMax=[]  UintegralTsProdOutMin=[]  UintegralTsProdOutMax=[]  UngainTsProdOutMin=[]  UngainTsProdOutMax=[]  ClampingZeroOutDataTypeStr=Inherit: Inherit via back propagation  ClampingZeroOutMin=[]  ClampingZeroOutMax=[]  FilterDenConstantOutDataTypeStr=Inherit: Inherit via back propagation  FilterDenConstantOutMin=[]  FilterDenConstantOutMax=[]  PCopyOutDataTypeStr=Inherit: Inherit via back propagation  PCopyOutMin=[]  PCopyOutMax=[]  NCopyOutDataTypeStr=Inherit: Inherit via back propagation  NCopyOutMin=[]  NCopyOutMax=[]  IntegratorContinuousStateAttributes=''  IntegratorStateMustResolveToSignalObject=off  IntegratorRTWStateStorageClass=Auto  FilterContinuousStateAttributes=''  FilterStateMustResolveToSignalObject=off  FilterRTWStateStorageClass=Auto  ParallelPVariant=InternalParameters  IdealPVariant=Disabled  IVariant=InternalParameters  DVariant=Disabled  IntegratorVariant=Continuous  SatVariant=Enabled  AWVariant=ContClampingParallel  PCopyVariant=Disabled  TRVariant=Disabled  FdbkBlocksVariant=Forward  IdealPFdbkVariant=Disabled  SatFdbkVariant=Disabled  DerivativeFilterVariant=Disabled  NVariant=Disabled  NCopyVariant=Disabled_SignalSpec  FilterICVariant=Disabled  IntegratorICVariant=InternalICs  ExternalResetVariant=Disabled  TRSumVariant=Passthrough  SumFdbkVariant=Disabled  SumVariant=Sum_PI  TsampFilterVariant=InternalTs  TsampNgainVariant=Passthrough  TsampIntegralVariant=Disabled_SignalSpec  ExternalSaturationOutDataTypeStr=Inherit: Same as second input  DerivativeSourceVariant=Disabled  PreIntVariant=InternalPreInt
  Rotor Torque : PMIOPort  Side=Left
  Rotor Anglular Velocity : PMIOPort  Port=2  Side=Left
  Voltage + : PMIOPort  Port=3  Side=Left
  Voltage - : PMIOPort  Port=4  Side=Left
  Angluar Velocity : Outport
  wires:
  w_cmd/1 -> Sum/1  "w_cmd"
  Sum/1 -> Thrust Controller/1  "w_e"
  PS-Simulink Converter4/1 -> Sum/2, Angluar Velocity/1  "w"
  Thrust Controller/1 -> Simulink-PS Converter/1  "w_controlled"
  connections:
  Rotational Multibody Interface/RConn1 -- Rotor Anglular Velocity/RConn1
  Motor 1/RConn3 -- Mechanical Rotational Reference1/LConn1
  Motor 1/LConn3 -- Rotational Multibody Interface/RConn2
  Rotational Multibody Interface/LConn1 -- Rotor Torque/RConn1
  Motor 1/RConn1 -- Voltage -/RConn1
  Mechanical Rotational Reference/LConn1 -- Rotational Multibody Interface/LConn2
  Motor 1/RConn2 -- PS-Simulink Converter4/LConn1
  Simulink-PS Converter/RConn1 -- Motor 1/LConn2
  Voltage +/RConn1 -- Motor 1/LConn1
